simulink model "open_loop"  (R2026b)
settings: Solver=FixedStepAuto  StopTime=10  EnableMultiTasking=on
undefined symbols (not defined in the file): Bambient, k, R_coil_ref, Vmax
libraries: stm32blockslib x4, stm32f4xxblockslib x2, stm32g4xxblockslib x2
settings Model: STM32="{\"DigitalPortRead\":{\"ID\":\"267\"},\"PWMOutput\":{\"ID\":\"274\"},\"TimerCapture\":[{\"ID\":\"277\"},{\"ID\":\"278\"},{\"ID\":\"279\"},{\"ID\":\"280\"}],\"HardwareInterrupt\":[{\"ID\":\"302\"},{\"ID\":\"315\"}]}"  Creator=Samuel  LastModifiedBy=Samuel
settings SolverCC: AutoInsertRateTranBlk=on
settings OptimizationCC: DefaultParameterBehavior=Inlined  DifferentSizesBufferReuse=on  EfficientTunableParamExpr=on  EnhancedBackFolding=on  MaxStackSize=512  OptimizationCustomize=off  OptimizeBlockOrder=speed  PassReuseOutputArgsAs=Individual arguments  RemoveInternalMemoryZeroInit=on  RemoveRootLevelIOMemoryZeroInit=on
settings DebuggingCC: ParameterTunabilityLossMsg=error
settings HardwareCC: ProdHWDeviceType=ARM Compatible->ARM Cortex-M  ProdLargestAtomicFloat=Double  ProdLargestAtomicInteger=Long  ProdLongLongMode=on
settings SFSimCC: MATLABDynamicMemAlloc=off
settings RTWCC: BuildConfiguration=Faster Runs  Description=Embedded Coder  HardwareBoard=STM32G4xx Based  SystemTargetFile=ert.tlc  TLCOptions=-aInlineSetEventsForThisBaseRateFcn=TLC_FALSE -aSuppressMultiTaskScheduler=TLC_FALSE -aRateBasedStepFcn=1  TemplateMakefile=ert_default_tmf  Toolchain=GNU Tools for STM32
settings CodeAppCC: ForceParamTrailComments=on  IgnoreCustomStorageClasses=off  InsertBlockDesc=on  OperatorAnnotations=on  SFDataObjDesc=on  SimulinkDataObjDesc=on
settings ERTTargetCC: CodeReplacementLibrary=ARM Cortex-M  CombineSignalStateStructs=on  ExtModeIntrfLevel=Level2 - Open  ExtModeMexFile=ext_xcp  ExtModeStaticAlloc=on
settings SimscapeCC: SimscapeUseEnergyAccounting=off

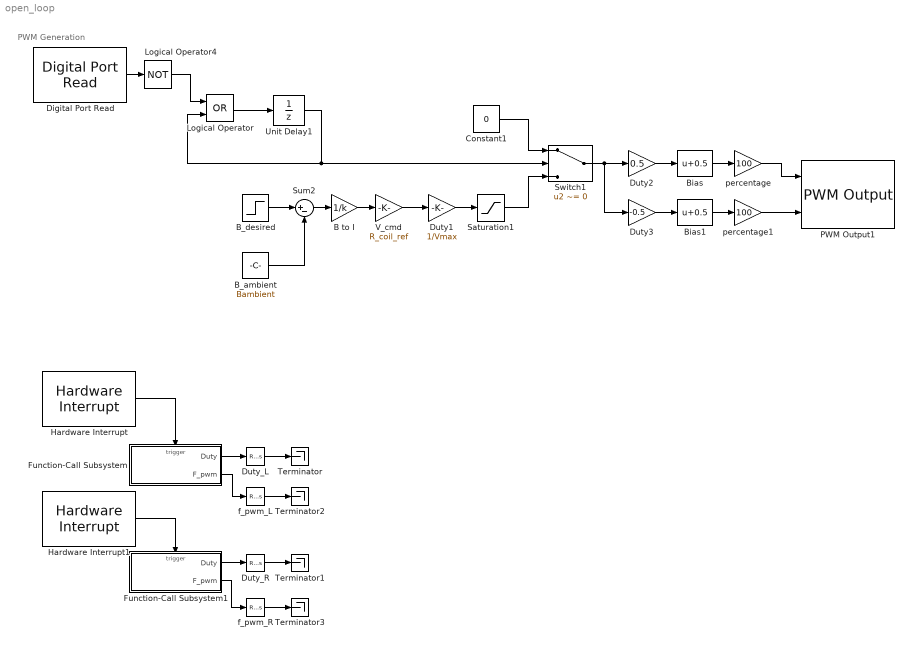
== system open_loop ==
  note: PWM Generation
  B to I : Gain  Gain=1/k
  B_ambient : Constant  Value=Bambient  SampleTime=1e-3
  B_desired : Step  Time=2  FinalValue=-100e-6  SampleTime=1e-3
  Bias : Bias  Bias=0.5  SaturateOnIntegerOverflow=off
  Bias1 : Bias  Bias=0.5  SaturateOnIntegerOverflow=off
  Constant1 : Constant  Value=0
  Digital Port Read : stm32f4xxblockslib/Digital Port Read  PortName=GPIOB  PinNumber=12  ReadOperation=on  IOAsArray=off  SampleTime=-1  EnableSimPort=off  hoistedMaskSrc=ECSoC/ECSimCodegen/Digital Port Read
      settings: LibrarySourceBlock=stm32g4xxblockslib/Digital Port Read
  Duty1 : Gain  Gain=1/Vmax
  Duty2 : Gain  Gain=0.5
  Duty3 : Gain  Gain=-0.5
  Duty_L : RateTransition  Deterministic=off  OutPortSampleTime=1e-3
  Duty_R : RateTransition  Deterministic=off  OutPortSampleTime=1e-3
  Function-Call Subsystem : Subsystem  TreatAsAtomicUnit=on
  Function-Call Subsystem1 : Subsystem  TreatAsAtomicUnit=on
  Hardware Interrupt : stm32g4xxblockslib/Hardware Interrupt  ISRGroup=Timer (TIM)  ISRName=TIM2_IRQHandler  ISRFunctionName=TIM2_IRQHandler  ISRNumber=43  TaskPriority=30  EventsList={ 'off', 'TIM2 Update', '1', 'inherit', 'off'; 'on', 'TIM2 CC1', '2', 'inherit', 'off'; 'off', 'TIM2 CC2', '3', 'inherit', 'off'; 'off', 'TIM2 CC3', '4', 'inherit', 'off'; 'off', 'TIM2 CC4', '5', 'inherit', 'off'; 'off', 'TIM2 Trigger', '6', 'inherit', 'off'; 'off', 'TIM2 DIR', '7', 'inherit', 'off'; 'off', 'TIM2 IDX', '8', 'inherit', 'off'; 'off', 'TIM2 IERR', '9', 'inherit', 'off'; 'off', 'TIM2 TERR', '10', 'inherit', 'off'; 'off', 'Custom event', '11', 'inherit', 'off' }  SelectedEvents={'TIM2 CC1'}  InternalTaskPriority=30  DisablePreemption=off  ClearInterruptFlagsAtEndOfEvent=off  InterruptDefinitionFile=$(TARGET_ROOT)/registry/interrupts/STM32F4xxBased_interrupts.xml  HardwareBoard=STM32G4xx Based  EnableSimPort=off
  Hardware Interrupt1 : stm32g4xxblockslib/Hardware Interrupt  ISRGroup=Timer (TIM)  ISRName=TIM3_IRQHandler  ISRFunctionName=TIM3_IRQHandler  ISRNumber=44  TaskPriority=31  EventsList={ 'off', 'TIM3 Update', '1', 'inherit', 'off'; 'on', 'TIM3 CC1', '2', 'inherit', 'off'; 'off', 'TIM3 CC2', '3', 'inherit', 'off'; 'off', 'TIM3 CC3', '4', 'inherit', 'off'; 'off', 'TIM3 CC4', '5', 'inherit', 'off'; 'off', 'TIM3 Trigger', '6', 'inherit', 'off'; 'off', 'TIM3 DIR', '7', 'inherit', 'off'; 'off', 'TIM3 IDX', '8', 'inherit', 'off'; 'off', 'TIM3 IERR', '9', 'inherit', 'off'; 'off', 'TIM3 TERR', '10', 'inherit', 'off'; 'off', 'Custom event', '11', 'inherit', 'off' }  SelectedEvents={'TIM3 CC1'}  InternalTaskPriority=31  DisablePreemption=off  ClearInterruptFlagsAtEndOfEvent=off  InterruptDefinitionFile=$(TARGET_ROOT)/registry/interrupts/STM32F4xxBased_interrupts.xml  HardwareBoard=STM32G4xx Based  EnableSimPort=off
  Logical Operator : Logic  Operator=OR  AllPortsSameDT=off  OutDataTypeStr=boolean
  Logical Operator4 : Logic  Operator=NOT  AllPortsSameDT=off  OutDataTypeStr=boolean
  PWM Output1 : stm32f4xxblockslib/PWM Output  ProcessorFamily=STM32G4  TimerModule=TIM1  DutycycleUnits=Percentage  EnableChannel1=on  EnableCaptureCompare1Input=off  EnableCaptureCompare1ComplementaryInput=off  EnableOutputCompare1ModeInput=off  EnableChannel2=on  EnableCaptureCompare2Input=off  EnableCaptureCompare2ComplementaryInput=off  EnableOutputCompare2ModeInput=off  EnableChannel3=off  EnableCaptureCompare3Input=off  EnableCaptureCompare3ComplementaryInput=off  EnableOutputCompare3ModeInput=off  EnableChannel4=off  EnableCaptureCompare4Input=off  EnableCaptureCompare4ComplementaryInput=off  EnableOutputCompare4ModeInput=off  EnableChannel5=off  EnableCaptureCompare5Input=off  EnableOutputCompare5ModeInput=off  EnableChannel6=off  EnableCaptureCompare6Input=off  EnableOutputCompare6ModeInput=off  EnableCounterInput=off  EnableMainOutputInput=off  EnableFrequencyInput=off  SetRCAfterCE=off  OutputDirection=off  OutputMainOutputEnableStatus=off  SampleTime=0.1  EnableSimPort=off  EnableUpdateEvent=off  EnableCaptureCompare1Event=off  EnableCaptureCompare2Event=off  EnableCaptureCompare3Event=off  EnableCaptureCompare4Event=off  EnableTriggerEvent=off  EnableBreakEvent=off  EnableBreakEvent2=off  hoistedMaskSrc=ECSoC/ECSimCodegen/PWM Output
      settings: LibrarySourceBlock=stm32g4xxblockslib/PWM Output
  Saturation1 : Saturate  UpperLimit=1  LowerLimit=-1
  Sum2 : Sum  Inputs=|+-
  Switch1 : Switch  Criteria=u2 ~= 0  SaturateOnIntegerOverflow=off  InputSameDT=off
  Terminator{,1..3} (4 alike) : Terminator
  Unit Delay1 : UnitDelay  SampleTime=1e-4
  V_cmd : Gain  Gain=R_coil_ref
  f_pwm_L : RateTransition  Deterministic=off  OutPortSampleTime=1e-3
  f_pwm_R : RateTransition  Deterministic=off  OutPortSampleTime=1e-3
  percentage : Gain  Gain=100
  percentage1 : Gain  Gain=100
  wires:
  B_desired/1 -> Sum2/1
  B_ambient/1 -> Sum2/2
  Sum2/1 -> B to I/1
  Logical Operator4/1 -> Logical Operator/1
  Digital Port Read/1 -> Logical Operator4/1
  Logical Operator/1 -> Unit Delay1/1
  Duty2/1 -> Bias/1
  Bias/1 -> percentage/1
  Switch1/1 -> Duty2/1, Duty3/1
  Unit Delay1/1 -> Logical Operator/2, Switch1/2
  Constant1/1 -> Switch1/1
  Saturation1/1 -> Switch1/3
  Duty1/1 -> Saturation1/1
  Duty3/1 -> Bias1/1
  Bias1/1 -> percentage1/1
  percentage/1 -> PWM Output1/1
  percentage1/1 -> PWM Output1/2
  B to I/1 -> V_cmd/1
  V_cmd/1 -> Duty1/1
  Function-Call Subsystem/1(Duty) -> Duty_L/1
  Function-Call Subsystem1/1(Duty) -> Duty_R/1
  Hardware Interrupt/1 -> Function-Call Subsystem/Trigger
  Hardware Interrupt1/1 -> Function-Call Subsystem1/Trigger
  Duty_L/1 -> Terminator/1
  Duty_R/1 -> Terminator1/1
  f_pwm_L/1 -> Terminator2/1
  Function-Call Subsystem/2(F_pwm) -> f_pwm_L/1
  f_pwm_R/1 -> Terminator3/1
  Function-Call Subsystem1/2(F_pwm) -> f_pwm_R/1

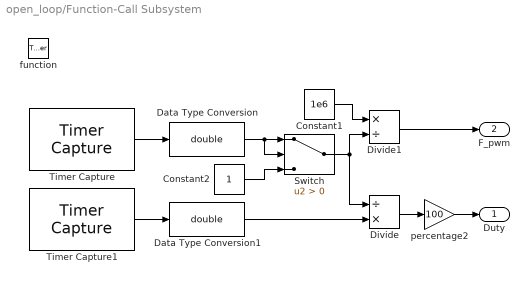
== system open_loop/Function-Call Subsystem ==
  function : TriggerPort  TriggerType=function-call  VariantControl=(inherit)
  Constant1 : Constant  Value=1e6
  Constant2 : Constant
  Data Type Conversion : DataTypeConversion  OutDataTypeStr=double  SaturateOnIntegerOverflow=off  RndMeth=Floor
  Data Type Conversion1 : DataTypeConversion  OutDataTypeStr=double  SaturateOnIntegerOverflow=off  RndMeth=Floor
  Divide : Product  Inputs=/*
  Divide1 : Product  Inputs=*/
  Switch : Switch  Criteria=u2 > Threshold  SaturateOnIntegerOverflow=off  InputSameDT=off
  Timer Capture : stm32blockslib/Timer Capture  TimerModule=TIM2  SelectedChannel=CH1  CaptureLength=1  OutputDataLength=off  OutputOverrunStatus=off  OutputDirection=off  SampleTime=-1
      settings: LibrarySourceBlock=stm32g4xxblockslib/Timer Capture
  Timer Capture1 : stm32blockslib/Timer Capture  TimerModule=TIM2  SelectedChannel=CH2  CaptureLength=1  OutputDataLength=off  OutputOverrunStatus=off  OutputDirection=off  SampleTime=-1
      settings: LibrarySourceBlock=stm32g4xxblockslib/Timer Capture
  percentage2 : Gain  Gain=100
  Duty : Outport
  F_pwm : Outport  Port=2
  wires:
  percentage2/1 -> Duty/1
  Switch/1 -> Divide1/2, Divide/1
  Data Type Conversion1/1 -> Divide/2
  Data Type Conversion/1 -> Switch/1, Switch/2
  Timer Capture1/1 -> Data Type Conversion1/1
  Constant2/1 -> Switch/3
  Timer Capture/1 -> Data Type Conversion/1
  Divide/1 -> percentage2/1
  Constant1/1 -> Divide1/1
  Divide1/1 -> F_pwm/1

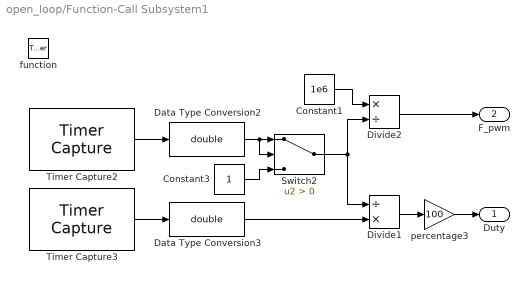
== system open_loop/Function-Call Subsystem1 ==
  function : TriggerPort  TriggerType=function-call  VariantControl=(inherit)
  Constant1 : Constant  Value=1e6
  Constant3 : Constant
  Data Type Conversion2 : DataTypeConversion  OutDataTypeStr=double  SaturateOnIntegerOverflow=off  RndMeth=Floor
  Data Type Conversion3 : DataTypeConversion  OutDataTypeStr=double  SaturateOnIntegerOverflow=off  RndMeth=Floor
  Divide1 : Product  Inputs=/*
  Divide2 : Product  Inputs=*/
  Switch2 : Switch  Criteria=u2 > Threshold  SaturateOnIntegerOverflow=off  InputSameDT=off
  Timer Capture2 : stm32blockslib/Timer Capture  TimerModule=TIM3  SelectedChannel=CH1  CaptureLength=1  OutputDataLength=off  OutputOverrunStatus=off  OutputDirection=off  SampleTime=-1
      settings: LibrarySourceBlock=stm32g4xxblockslib/Timer Capture
  Timer Capture3 : stm32blockslib/Timer Capture  TimerModule=TIM3  SelectedChannel=CH2  CaptureLength=1  OutputDataLength=off  OutputOverrunStatus=off  OutputDirection=off  SampleTime=-1
      settings: LibrarySourceBlock=stm32g4xxblockslib/Timer Capture
  percentage3 : Gain  Gain=100
  Duty : Outport
  F_pwm : Outport  Port=2
  wires:
  percentage3/1 -> Duty/1
  Data Type Conversion2/1 -> Switch2/2, Switch2/1
  Timer Capture2/1 -> Data Type Conversion2/1
  Switch2/1 -> Divide2/2, Divide1/1
  Constant3/1 -> Switch2/3
  Divide1/1 -> percentage3/1
  Timer Capture3/1 -> Data Type Conversion3/1
  Data Type Conversion3/1 -> Divide1/2
  Constant1/1 -> Divide2/1
  Divide2/1 -> F_pwm/1
